simulink model "Simulink_ABS"  (R2026b)
settings: Solver=VariableStepAuto  StopTime=10  MaxStep=1e-3
InitFcn:
  | Code_ABS
values from neighbouring files (symbols this model uses):
  A = 4000    [Code_ABS.m]
  acc = -1/m    (= -0.001)    [Code_ABS.m]
  c_roues = N*rRoue    (= 735.75)    [Code_ABS.m]
  f_adh = 0.8    [Code_ABS.m]
  f_tab = [0 0.60 0.85 0.93 0.95 0.88 0.80 0.73 0.68 0.63 0.60]    [Code_ABS.m]
  gliss_tab = [0 0.05 0.10 0.15 0.20 0.30 0.40 0.50 0.60 0.80 1.00]    [Code_ABS.m]
  J = 0.5    [Code_ABS.m]
  N = m*g0/4    (= 2452.5)    [Code_ABS.m]
  rRoue = 0.3    [Code_ABS.m]
  v0 = 27.77    [Code_ABS.m]
libraries: simulink x2
settings Model: Creator=Tom  LastModifiedBy=Tom

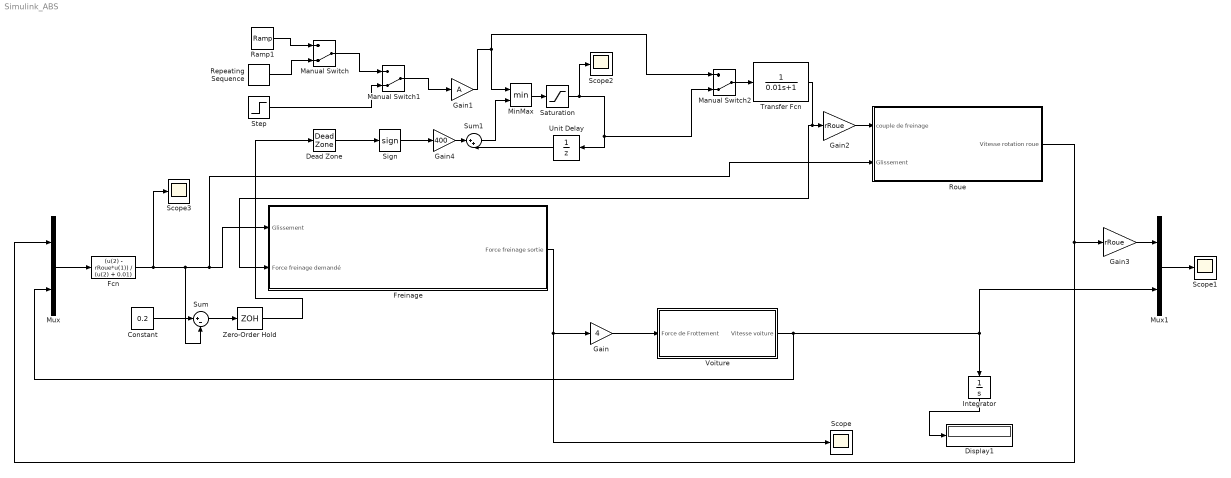
== system Simulink_ABS ==
  Constant : Constant  Value=0.2
  Dead Zone : DeadZone  LowerValue=-0.01  UpperValue=0.01
  Display1 : Display
  Fcn : Fcn  Expr=(u(2) - rRoue*u(1)) / (u(2) + 0.01)
  Freinage : Subsystem
  Gain : Gain  Gain=4
  Gain1 : Gain  Gain=A
  Gain2 : Gain  Gain=rRoue
  Gain3 : Gain  Gain=rRoue
  Gain4 : Gain  Gain=400
  Integrator : Integrator
  Manual Switch : ManualSwitch  CurrentSetting=0
  Manual Switch1 : ManualSwitch  CurrentSetting=0
  Manual Switch2 : ManualSwitch  CurrentSetting=0
  MinMax : MinMax  Inputs=2
  Mux : Mux  Inputs=2
  Mux1 : Mux  Inputs=2
  Ramp1 : simulink/Sources/Ramp  slope=1000  start=0  InitialOutput=0
  Repeating Sequence : simulink/Sources/Repeating Sequence  rep_seq_t=[0 1 8 9 10]  rep_seq_y=[0 1 1 0 0]
  Roue : Subsystem
  Saturation : Saturate  UpperLimit=inf  LowerLimit=0
  Scope{,1..3} (4 alike) : Scope
      Scope settings: ActiveDisplayYMinimum=471.5  ActiveDisplayYMaximum=2471.5
      Scope1 settings: ActiveDisplayYMinimum=-11.570833333333331  ActiveDisplayYMaximum=104.13749999999999
      Scope2 settings: ActiveDisplayYMinimum=2388.1770780684733  ActiveDisplayYMaximum=2539.2393617203752  DataLoggingVariableName=ScopeData2
      Scope3 settings: ActiveDisplayYMinimum=0.11711730188145665  ActiveDisplayYMaximum=0.18650673751599733  DataLoggingVariableName=ScopeData3
  Sign : Signum
  Step : Step  Time=0  SampleTime=0
  Sum : Sum  Inputs=|+-
  Sum1 : Sum  Inputs=|++
  Transfer Fcn : TransferFcn  Denominator=[0.01 1]
  Unit Delay : UnitDelay  SampleTime=1e-4
  Voiture : Subsystem
  Zero-Order Hold : ZeroOrderHold  SampleTime=1e-4
  wires:
  Gain/1 -> Voiture/1(Force de Frottement)
  Ramp1/1 -> Manual Switch/1
  Repeating Sequence/1 -> Manual Switch/2
  Step/1 -> Manual Switch1/2
  Manual Switch/1 -> Manual Switch1/1
  Manual Switch1/1 -> Gain1/1
  Gain1/1 -> Manual Switch2/1, MinMax/1
  Gain2/1 -> Roue/1(couple de freinage)
  Roue/1(Vitesse rotation roue) -> Gain3/1, Mux/1
  Mux/1 -> Fcn/1
  Fcn/1 -> Scope3/1, Sum/2, Roue/2(Glissement), Freinage/1(Glissement)
  Freinage/1(Force freinage sortie) -> Scope/1, Gain/1
  Voiture/1(Vitesse voiture) -> Mux1/2, Integrator/1, Mux/2
  Integrator/1 -> Display1/1
  Mux1/1 -> Scope1/1
  Gain3/1 -> Mux1/1
  Transfer Fcn/1 -> Freinage/2(Force freinage demandé), Gain2/1
  Constant/1 -> Sum/1
  Zero-Order Hold/1 -> Dead Zone/1
  MinMax/1 -> Saturation/1
  Manual Switch2/1 -> Transfer Fcn/1
  Sum/1 -> Zero-Order Hold/1
  Sign/1 -> Gain4/1
  Gain4/1 -> Sum1/1
  Sum1/1 -> MinMax/2
  Saturation/1 -> Scope2/1, Manual Switch2/2, Unit Delay/1
  Unit Delay/1 -> Sum1/2
  Dead Zone/1 -> Sign/1

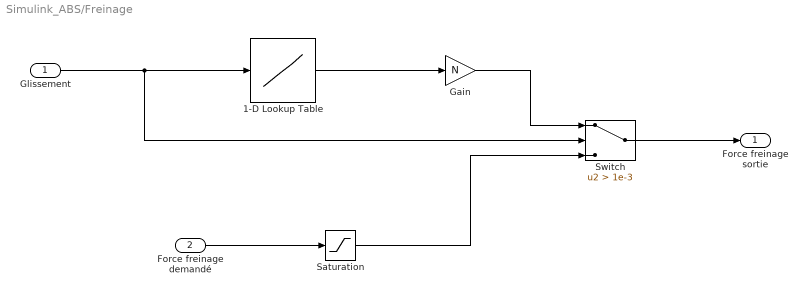
== system Simulink_ABS/Freinage ==
  Glissement : Inport
  Force freinage demandé : Inport  Port=2
  1-D Lookup Table : Lookup_n-D  NumberOfTableDimensions=1  BreakpointsForDimension1=gliss_tab  Table=f_tab  InternalRulePriority=Speed  RndMeth=Simplest
  Gain : Gain  Gain=N
  Saturation : Saturate  UpperLimit=f_adh*N  LowerLimit=0
  Switch : Switch  Criteria=u2 > Threshold  Threshold=1e-3  SaturateOnIntegerOverflow=off  InputSameDT=off
  Force freinage sortie : Outport
  wires:
  Force freinage demandé/1 -> Saturation/1
  Gain/1 -> Switch/1
  1-D Lookup Table/1 -> Gain/1
  Glissement/1 -> 1-D Lookup Table/1, Switch/2
  Switch/1 -> Force freinage sortie/1
  Saturation/1 -> Switch/3

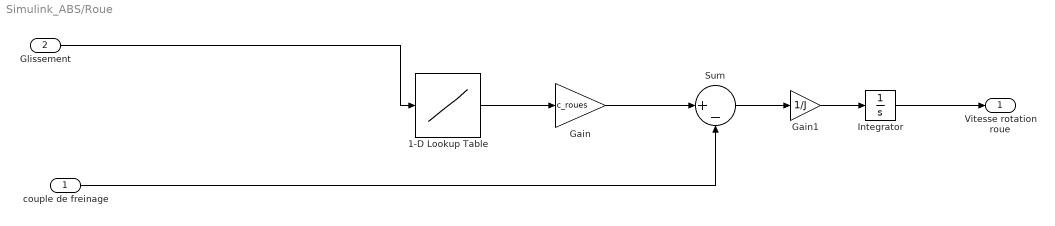
== system Simulink_ABS/Roue ==
  couple de freinage : Inport
  Glissement : Inport  Port=2
  1-D Lookup Table : Lookup_n-D  NumberOfTableDimensions=1  BreakpointsForDimension1=gliss_tab  Table=f_tab  InternalRulePriority=Speed  RndMeth=Simplest
  Gain : Gain  Gain=c_roues
  Gain1 : Gain  Gain=1/J
  Integrator : Integrator  InitialCondition=v0/rRoue  LimitOutput=on  LowerSaturationLimit=0
  Sum : Sum  Inputs=|+-
  Vitesse rotation roue : Outport
  wires:
  1-D Lookup Table/1 -> Gain/1
  Gain/1 -> Sum/1
  Gain1/1 -> Integrator/1
  Glissement/1 -> 1-D Lookup Table/1
  Sum/1 -> Gain1/1
  Integrator/1 -> Vitesse rotation roue/1
  couple de freinage/1 -> Sum/2

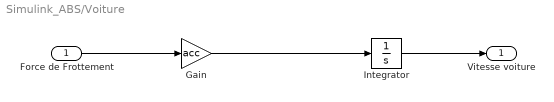
== system Simulink_ABS/Voiture ==
  Force de Frottement : Inport
  Gain : Gain  Gain=acc
  Integrator : Integrator  InitialCondition=v0  LimitOutput=on  LowerSaturationLimit=0
  Vitesse voiture : Outport
  wires:
  Gain/1 -> Integrator/1
  Force de Frottement/1 -> Gain/1
  Integrator/1 -> Vitesse voiture/1
